simulink model "TOAD_Simulation_CPP"  (R2026a)
settings: Solver=VariableStepAuto  StopTime=50
values from neighbouring files (symbols this model uses):
  bGrom = G.C / (2 * sqrt(kGrom * m_FC))    [LoadTOADSim.m]
  constants6DoF = LoadTOADParams(Vehicle)    [LoadTOADSim.m]
  dt_SIM = 1/500    (= 0.002)    [LoadTOADSim.m]
  G_RMAX = 4    [LoadTOADSim.m]
  highEnd = 800    [LoadTOADSim.m]
  IMU_Rate = 500    [LoadTOADSim.m]
  Kg2 = 0.03    [LoadTOADSim.m]
  kGrom = G.K    [LoadTOADSim.m]
  lowEnd = 50    [LoadTOADSim.m]
  magDistMatrix = [dM_xx, dM_xy, dM_xz ... (first row only)    [LoadTOADSim.m]
  x0 = [1; zeros(12,1); constants6DoF.OxMass; constants6DoF.FuMass]    [LoadTOADSim.m]
undefined symbols (not defined in the file or in its folder): DiscIntNeverNeededParam, dt
libraries: aerolibnav x2, simulink x2
settings Model: PacingRate=0.890000  Creator=antho  LastModifiedBy=pplat

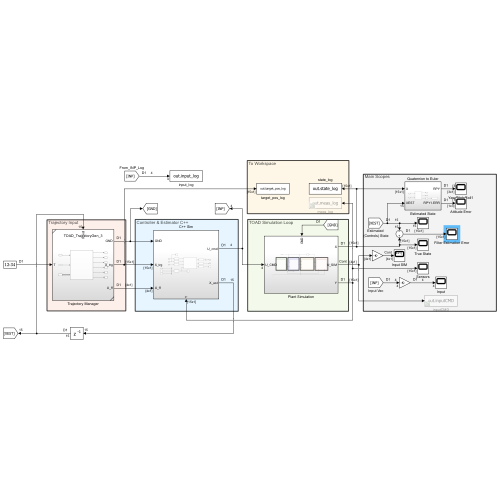
[thumbnail: Simulink's stored preview of the top-level diagram]
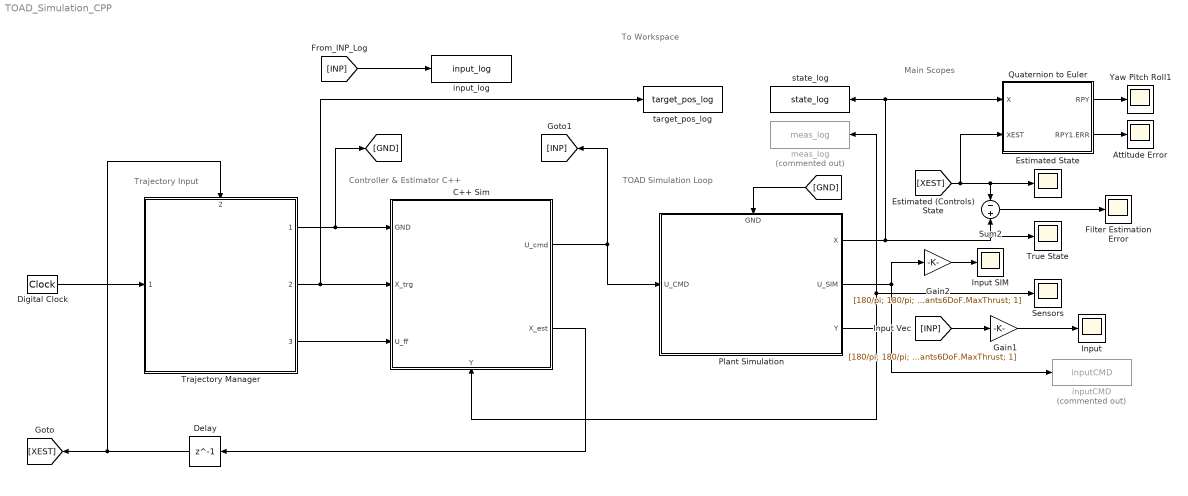
== system TOAD_Simulation_CPP ==
  note: To Workspace
  note: Main Scopes
  note: Trajectory Input
  note: Controller & Estimator C++
  note: TOAD Simulation Loop
  Attitude Error : Scope
      settings: ActiveDisplayYMinimum=-2.8585138814503157  ActiveDisplayYMaximum=11.108081672047327  DataLoggingVariableName=ScopeData9
  C++ Sim : Subsystem
      settings: PortSchema="{\"entries\":[{\"content\":{\"sides\":[{\"content\":{\"connectorIds\":[\"In1\",\"In2\",\"In3\"]},\"type\":\"ConnectorPlacement.EquallySpacedRectSide\",\"uuid\":\"4671e83a-8ca8-4575-bcdb-bf09507d43ac\"},{\"content\":{\"connectorIds\":[\"Out1\",\"Out2\"],\"side\":\"RIGHT\"},\"type\":\"ConnectorPlacement.EquallySpacedRectSide\",\"uuid\":\"a3e587af-0321-4bb5-b0a1-9da4dd43c686\"},{\"content\":{\"side\":\"TOP\"},\"type\":\"ConnectorPlacement.EquallySpacedRectSide\",\"uuid\":\"4e506283-964c-4194-bd88-e6573f16e4a7\"},{\"content\":{\"connectorIds\":[\"In4\"],\"side\":\"BOTTOM\"},\"type\":\"ConnectorPlacement.EquallySpacedRectSide\",\"uuid\":\"96ffffcd-a794-471a-8d82-32f73f1e6258\"}]},\"type\":\"ConnectorPlacement.EquallySpacedConnector\",\"uuid\":\"7e610c41-1f3b-432e-89ab-1ded86d82775\"}],\"packageUris\":[\"http://schema.mathworks.com/mf0/Connector/R2020b\"],\"version\":\"1.0\"}"
  Delay : Delay  DelayLength=1  InitialCondition=[1; zeros(14,1)]
  Digital Clock : DigitalClock  SampleTime=dt_SIM
  Estimated State : Scope
      settings: ActiveDisplayYMinimum=-0.79048423235500387  ActiveDisplayYMaximum=0.44471004558217864
  Filter Estimation Error : Scope
      settings: ActiveDisplayYMinimum=-0.43763268691917351  ActiveDisplayYMaximum=0.34444045907476623  DataLoggingVariableName=ScopeData2
  Gain1 : Gain  Gain=[180/pi; 180/pi; 1 / constants6DoF.MaxThrust; 1]
  Gain2 : Gain  Gain=[180/pi; 180/pi; 1 / constants6DoF.MaxThrust; 1]
  Input : Scope
      settings: ActiveDisplayYMinimum=-2.2667092424589841  ActiveDisplayYMaximum=2.729210355412238  DataLoggingVariableName=ScopeData6
  Input SIM : Scope
      settings: ActiveDisplayYMinimum=-2.0167562812566757  ActiveDisplayYMaximum=7.29010234773159  DataLoggingVariableName=ScopeData4
  Plant Simulation : Subsystem
      settings: PortSchema="{\"entries\":[{\"content\":{\"sides\":[{\"content\":{\"connectorIds\":[\"In1\"]},\"type\":\"ConnectorPlacement.EquallySpacedRectSide\",\"uuid\":\"1e23e861-4363-4f64-8b24-83286696985d\"},{\"content\":{\"connectorIds\":[\"Out1\",\"Out2\",\"Out3\"],\"side\":\"RIGHT\"},\"type\":\"ConnectorPlacement.EquallySpacedRectSide\",\"uuid\":\"b75b2d72-241b-467f-aafa-6008c8f1cd07\"},{\"content\":{\"connectorIds\":[\"In2\"],\"side\":\"TOP\"},\"type\":\"ConnectorPlacement.EquallySpacedRectSide\",\"uuid\":\"dda51a79-77a4-44ba-8754-0dda6b153588\"}]},\"type\":\"ConnectorPlacement.EquallySpacedConnector\",\"uuid\":\"1bd609f5-eeaa-4870-8a50-1642b8d6b239\"}],\"packageUris\":[\"http://schema.mathworks.com/mf0/Connector/R2020b\"],\"version\":\"1.0\"}"
  Quaternion to Euler : Subsystem
  Sensors : Scope
      settings: ActiveDisplayYMinimum=-0.86115231127145009  ActiveDisplayYMaximum=0.76236237160727249  DataLoggingVariableName=ScopeData3
  Sum2 : Sum  Inputs=-|+
  Trajectory Manager : Subsystem  ReferencedSubsystem=TOAD_TrajectoryGen_3
      settings: PortSchema="{\"entries\":[{\"content\":{\"sides\":[{\"content\":{\"connectorIds\":[\"In1\"]},\"type\":\"ConnectorPlacement.EquallySpacedRectSide\",\"uuid\":\"53aeece0-39f7-4f67-ba76-7d162a9bdc19\"},{\"content\":{\"connectorIds\":[\"Out1\",\"Out2\",\"Out3\"],\"side\":\"RIGHT\"},\"type\":\"ConnectorPlacement.EquallySpacedRectSide\",\"uuid\":\"ed850121-4575-4d77-9468-bb12120e9ba8\"},{\"content\":{\"connectorIds\":[\"In2\"],\"side\":\"TOP\"},\"type\":\"ConnectorPlacement.EquallySpacedRectSide\",\"uuid\":\"a0a50c51-23a8-460d-b4f4-86ce8b2346c6\"}]},\"type\":\"ConnectorPlacement.EquallySpacedConnector\",\"uuid\":\"ca42ea5e-ce10-4bee-86cd-a79e465aaa56\"}],\"packageUris\":[\"http://schema.mathworks.com/mf0/Connector/R2020b\"],\"version\":\"1.0\"}"
  True State : Scope
      settings: ActiveDisplayYMinimum=-0.82145720567291391  ActiveDisplayYMaximum=0.0015477167542865544
  Yaw Pitch Roll1 : Scope
      settings: ActiveDisplayYMinimum=-35.86119806852372  ActiveDisplayYMaximum=29.416743225810393  DataLoggingVariableName=ScopeData5
  inputCMD : ToWorkspace  Commented=on  VariableName=inputCMD  SaveFormat=Timeseries  SampleTime=-1
  input_log : ToWorkspace  VariableName=input_log  SaveFormat=Timeseries  SampleTime=0.02
  meas_log : ToWorkspace  Commented=on  VariableName=meas_log  SaveFormat=Timeseries  SampleTime=-1
  state_log : ToWorkspace  VariableName=state_log  SaveFormat=Timeseries  SampleTime=0.02
  target_pos_log : ToWorkspace  VariableName=target_pos_log  SaveFormat=Timeseries  SampleTime=0.02
  wires:
  Digital Clock/1 -> Trajectory Manager/1
  [XEST] -> Estimated State/1, Sum2/1, Quaternion to Euler/2(XEST)
  Sum2/1 -> Filter Estimation Error/1
  Trajectory Manager/1 -> [GND], C++ Sim/1(GND)
  [INP] -> Gain1/1
  Gain1/1 -> Input/1
  Gain2/1 -> Input SIM/1
  Plant Simulation/2(U_SIM) -> Gain2/1, inputCMD/1
  Plant Simulation/3(Y) -> C++ Sim/4(Y), meas_log/1, Sensors/1
  Plant Simulation/1(X) -> state_log/1, Quaternion to Euler/1(X), Sum2/2, True State/1
  Delay/1 -> Trajectory Manager/2, [XEST]
  Trajectory Manager/2 -> target_pos_log/1, C++ Sim/2(X_trg)
  Quaternion to Euler/1(RPY) -> Yaw Pitch Roll1/1
  Quaternion to Euler/2(RPY1.ERR) -> Attitude Error/1
  [GND] -> Plant Simulation/2(GND)
  [INP] -> input_log/1
  C++ Sim/1(U_cmd) -> Plant Simulation/1(U_CMD), [INP]
  Trajectory Manager/3 -> C++ Sim/3(U_ff)
  C++ Sim/2(X_est) -> Delay/1

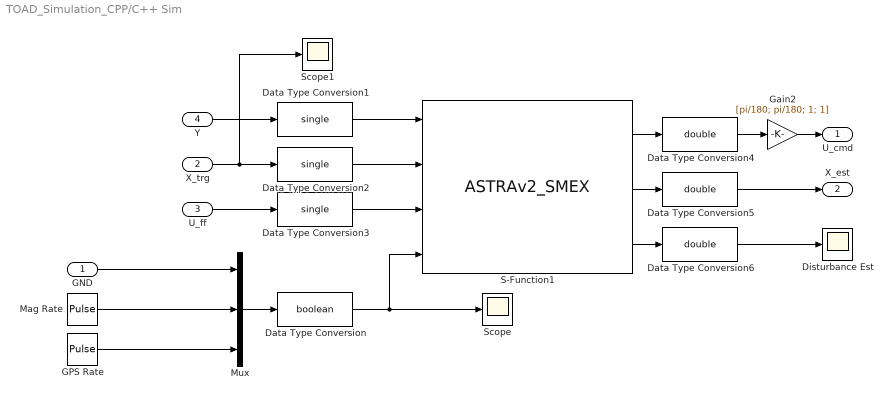
== system TOAD_Simulation_CPP/C++ Sim ==
  GND : Inport
  X_trg : Inport  Port=2
  U_ff : Inport  Port=3
  Y : Inport  Port=4
  Data Type Conversion : DataTypeConversion  OutDataTypeStr=boolean  SaturateOnIntegerOverflow=off  RndMeth=Floor
  Data Type Conversion1 : DataTypeConversion  OutDataTypeStr=single  SaturateOnIntegerOverflow=off  RndMeth=Floor
  Data Type Conversion2 : DataTypeConversion  OutDataTypeStr=single  SaturateOnIntegerOverflow=off  RndMeth=Floor
  Data Type Conversion3 : DataTypeConversion  OutDataTypeStr=single  SaturateOnIntegerOverflow=off  RndMeth=Floor
  Data Type Conversion4 : DataTypeConversion  OutDataTypeStr=double  SaturateOnIntegerOverflow=off  RndMeth=Floor
  Data Type Conversion5 : DataTypeConversion  OutDataTypeStr=double  SaturateOnIntegerOverflow=off  RndMeth=Floor
  Data Type Conversion6 : DataTypeConversion  OutDataTypeStr=double  SaturateOnIntegerOverflow=off  RndMeth=Floor
  Disturbance Est : Scope
      settings: ActiveDisplayYMinimum=-1  ActiveDisplayYMaximum=1  DataLoggingVariableName=ScopeData8
  GPS Rate : DiscretePulseGenerator  Period=50  SampleTime=dt_SIM
  Gain2 : Gain  Gain=[pi/180; pi/180; 1; 1]
  Mag Rate : DiscretePulseGenerator  Period=4  SampleTime=dt_SIM
  Mux : Mux  Inputs=3
  S-Function1 : S-Function  FunctionName=ASTRAv2_SMEX  SFunctionDeploymentMode=off  EnableBusSupport=off
  Scope : Scope
      settings: ActiveDisplayYMinimum=-0.12499999999999997  ActiveDisplayYMaximum=1.125  DataLoggingVariableName=ScopeData7
  Scope1 : Scope
      settings: ActiveDisplayYMinimum=-1  ActiveDisplayYMaximum=1  DataLoggingVariableName=ScopeData11
  U_cmd : Outport
  X_est : Outport  Port=2
  wires:
  S-Function1/2 -> Data Type Conversion5/1
  Y/1 -> Data Type Conversion1/1
  X_trg/1 -> Scope1/1, Data Type Conversion2/1
  S-Function1/1 -> Data Type Conversion4/1
  U_ff/1 -> Data Type Conversion3/1
  GND/1 -> Mux/1
  Mux/1 -> Data Type Conversion/1
  Mag Rate/1 -> Mux/2
  GPS Rate/1 -> Mux/3
  Data Type Conversion/1 -> Scope/1, S-Function1/4
  Data Type Conversion1/1 -> S-Function1/1
  Data Type Conversion2/1 -> S-Function1/2
  Data Type Conversion3/1 -> S-Function1/3
  Data Type Conversion4/1 -> Gain2/1
  Data Type Conversion5/1 -> X_est/1
  Gain2/1 -> U_cmd/1
  Data Type Conversion6/1 -> Disturbance Est/1
  S-Function1/3 -> Data Type Conversion6/1

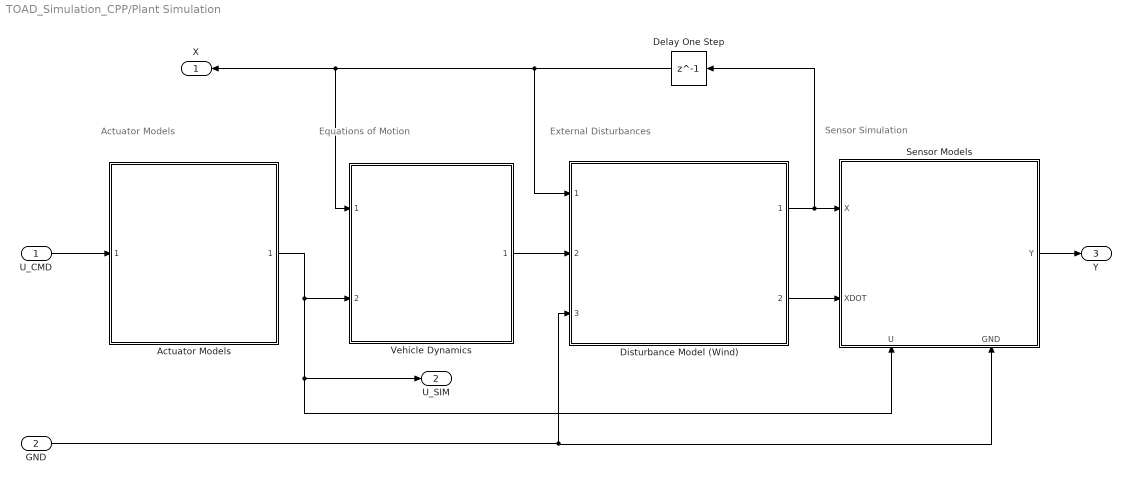
== system TOAD_Simulation_CPP/Plant Simulation ==
  note: Equations of Motion
  note: Actuator Models
  note: External Disturbances
  note: Sensor Simulation
  U_CMD : Inport
  GND : Inport  Port=2
  Actuator Models : Subsystem  ReferencedSubsystem=Actuator_Models_2
  Delay One Step : Delay  DelayLength=1  InitialCondition=x0
  Disturbance Model (Wind) : Subsystem  ReferencedSubsystem=Dist_Models_Integrator_2
  Sensor Models : Subsystem
      settings: PortSchema="{\"entries\":[{\"content\":{\"sides\":[{\"content\":{\"connectorIds\":[\"In1\",\"In2\"]},\"type\":\"ConnectorPlacement.EquallySpacedRectSide\",\"uuid\":\"9bc4a206-bba4-4c50-88a9-89b0392ab722\"},{\"content\":{\"connectorIds\":[\"Out1\"],\"side\":\"RIGHT\"},\"type\":\"ConnectorPlacement.EquallySpacedRectSide\",\"uuid\":\"162bbd17-e1b8-4f29-9191-53e17e38d79d\"},{\"content\":{\"side\":\"TOP\"},\"type\":\"ConnectorPlacement.EquallySpacedRectSide\",\"uuid\":\"c56a23db-6a5c-435f-99fd-d50fc9dbdc94\"},{\"content\":{\"connectorIds\":[\"In3\",\"In4\"],\"side\":\"BOTTOM\"},\"type\":\"ConnectorPlacement.EquallySpacedRectSide\",\"uuid\":\"e0c2a0dc-3b7a-40ac-8345-28e7bf7b9405\"}]},\"type\":\"ConnectorPlacement.EquallySpacedConnector\",\"uuid\":\"d1c29f55-9be5-4f45-9d70-06beba2c2f44\"}],\"packageUris\":[\"http://schema.mathworks.com/mf0/Connector/R2020b\"],\"version\":\"1.0\"}"
  Vehicle Dynamics : Subsystem  ReferencedSubsystem=Vehicle_Dynamics_2
  X : Outport
  U_SIM : Outport  Port=2
  Y : Outport  Port=3
  wires:
  Sensor Models/1(Y) -> Y/1
  Disturbance Model (Wind)/1 -> Delay One Step/1, Sensor Models/1(X)
  Disturbance Model (Wind)/2 -> Sensor Models/2(XDOT)
  Actuator Models/1 -> Vehicle Dynamics/2, U_SIM/1, Sensor Models/3(U)
  Vehicle Dynamics/1 -> Disturbance Model (Wind)/2
  U_CMD/1 -> Actuator Models/1
  GND/1 -> Disturbance Model (Wind)/3, Sensor Models/4(GND)
  Delay One Step/1 -> Disturbance Model (Wind)/1, Vehicle Dynamics/1, X/1

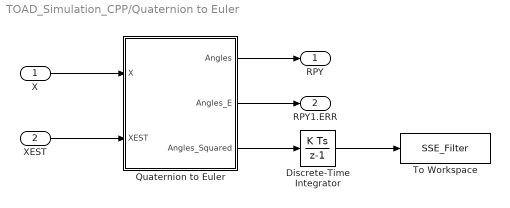
== system TOAD_Simulation_CPP/Quaternion to Euler ==
  X : Inport
  XEST : Inport  Port=2
  Discrete-Time Integrator : DiscreteIntegrator  InitialCondition=[0; 0; 0]'  SampleTime=-1  ICPrevOutput=DiscIntNeverNeededParam  ICPrevScaledInput=DiscIntNeverNeededParam
  Quaternion to Euler : MATLAB Function  TreatAsAtomicUnit=on
  To Workspace : ToWorkspace  VariableName=SSE_Filter  SampleTime=-1
      settings: MaxDataPoints=1
  RPY : Outport
  RPY1.ERR : Outport  Port=2
  wires:
  X/1 -> Quaternion to Euler/1(X)
  Quaternion to Euler/1(Angles) -> RPY/1
  XEST/1 -> Quaternion to Euler/2(XEST)
  Quaternion to Euler/2(Angles_E) -> RPY1.ERR/1
  Quaternion to Euler/3(Angles_Squared) -> Discrete-Time Integrator/1
  Discrete-Time Integrator/1 -> To Workspace/1

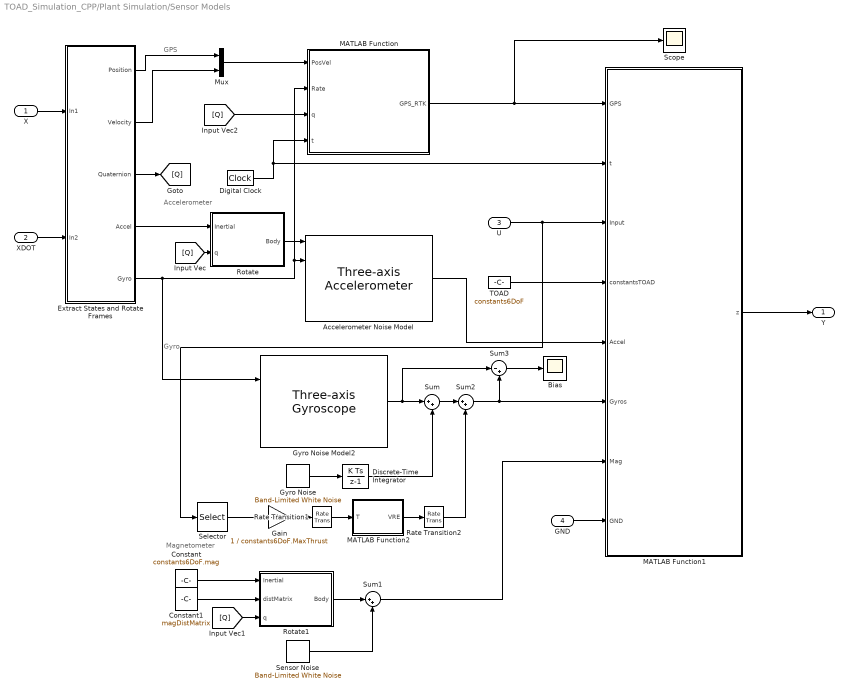
== system TOAD_Simulation_CPP/Plant Simulation/Sensor Models ==
  note: Gyro
  note: Accelerometer
  note: Magnetometer
  note: GPS
  X : Inport  PortDimensions=[15,1]
  XDOT : Inport  Port=2  PortDimensions=[15,1]
  U : Inport  Port=3
  GND : Inport  Port=4
  Accelerometer Noise Model : aerolibnav/Three-axis Accelerometer  units=Metric (MKS)  acc=[0 0 0.15]  gtype=on  dtype_a=on  w_a=190  z_a=0.707  a_sf_cc=eye(3)  a_bias=accelBias  a_Ts=1 / IMU_Rate  a_rand=on  a_seeds=[23093 23094 23095]  a_pow=ones(1,3) * 0.008^2 * 1 / IMU_Rate  a_sat="[-inf  -inf  -inf  inf inf inf]"
  Bias : Scope
      settings: ActiveDisplayYMinimum=-0.13135966855304979  ActiveDisplayYMaximum=1.1258739508928557  DataLoggingVariableName=ScopeData20
  Constant : Constant  Value=constants6DoF.mag
  Constant1 : Constant  Value=magDistMatrix
  Digital Clock : DigitalClock  SampleTime=dt_SIM
  Discrete-Time Integrator : DiscreteIntegrator  SampleTime=-1  ICPrevOutput=DiscIntNeverNeededParam  ICPrevScaledInput=DiscIntNeverNeededParam
  Extract States and Rotate Frames : Subsystem
  Gain : Gain  Gain=1 / constants6DoF.MaxThrust
  Gyro Noise : simulink/Sources/Band-Limited White Noise  Cov=gyroNoisePower  Ts=dt_SIM  seed=[23341,23342,23343]
  Gyro Noise Model2 : aerolibnav/Three-axis Gyroscope  dtype_g=on  w_g=190  z_g=0.707  g_sf_cc=eye(3)  g_bias=gyroBias  g_sen=0  g_Ts=1 / IMU_Rate  g_rand=on  g_seeds=[23093 23094 23095]  g_pow=ones(1,3) * 0.001^2 * dt  g_sat="[-inf  -inf  -inf  inf inf inf]"
  MATLAB Function : MATLAB Function  TreatAsAtomicUnit=on
  MATLAB Function1 : MATLAB Function  TreatAsAtomicUnit=on
  MATLAB Function2 : MATLAB Function  TreatAsAtomicUnit=on
  Mux : Mux  Inputs=2
  Rate Transition1 : RateTransition  InitialCondition=1  OutPortSampleTime=1/50
  Rate Transition2 : RateTransition  InitialCondition=1  OutPortSampleTime=dt_SIM
  Rotate : MATLAB Function  TreatAsAtomicUnit=on
  Rotate1 : MATLAB Function  TreatAsAtomicUnit=on
  Scope : Scope
      settings: ActiveDisplayYMinimum=-1  ActiveDisplayYMaximum=1  DataLoggingVariableName=ScopeData10
  Selector : Selector  IndexOptions=Index vector (dialog)  Indices=[3]  OutputSizes=1
  Sensor Noise : simulink/Sources/Band-Limited White Noise  Cov=(4E-4)^2  Ts=dt_SIM  seed=[23341,23342,23343]
  Sum : Sum  Inputs=|++
  Sum1 : Sum  Inputs=|++
  Sum2 : Sum  Inputs=|++
  Sum3 : Sum  Inputs=|-+
  TOAD : Constant  Value=constants6DoF  OutDataTypeStr=Bus: Vehicle_Bus
  Y : Outport
  wires:
  X/1 -> Extract States and Rotate Frames/1(In1)
  XDOT/1 -> Extract States and Rotate Frames/2(In2)
  Digital Clock/1 -> MATLAB Function/4(t), MATLAB Function1/2(t)
  Extract States and Rotate Frames/5(Gyro) -> Accelerometer Noise Model/2, MATLAB Function/2(Rate), Gyro Noise Model2/1
  Extract States and Rotate Frames/3(Quaternion) -> [Q]
  Rotate/1(Body) -> Accelerometer Noise Model/1
  Extract States and Rotate Frames/4(Accel) -> Rotate/1(Inertial)
  [Q] -> Rotate/2(q)
  Constant/1 -> Rotate1/1(Inertial)
  [Q] -> Rotate1/3(q)
  Sensor Noise/1 -> Sum1/2
  Rotate1/1(Body) -> Sum1/1
  Sum1/1 -> MATLAB Function1/7(Mag)
  MATLAB Function/1(GPS_RTK) -> Scope/1, MATLAB Function1/1(GPS)
  Accelerometer Noise Model/1 -> MATLAB Function1/5(Accel)
  Gyro Noise Model2/1 -> Sum3/1, Sum/1
  MATLAB Function1/1(z) -> Y/1
  TOAD/1 -> MATLAB Function1/4(constantsTOAD)
  Extract States and Rotate Frames/2(Velocity) -> Mux/2
  Mux/1 -> MATLAB Function/1(PosVel)
  Extract States and Rotate Frames/1(Position) -> Mux/1
  U/1 -> Selector/1, MATLAB Function1/3(Input)
  GND/1 -> MATLAB Function1/8(GND)
  Constant1/1 -> Rotate1/2(distMatrix)
  [Q] -> MATLAB Function/3(q)
  Gyro Noise/1 -> Discrete-Time Integrator/1
  Sum/1 -> Sum2/1
  Discrete-Time Integrator/1 -> Sum/2
  MATLAB Function2/1(VRE) -> Rate Transition2/1
  Sum2/1 -> MATLAB Function1/6(Gyros), Sum3/2
  Selector/1 -> Gain/1
  Gain/1 -> Rate Transition1/1
  Sum3/1 -> Bias/1
  Rate Transition1/1 -> MATLAB Function2/1(T)
  Rate Transition2/1 -> Sum2/2

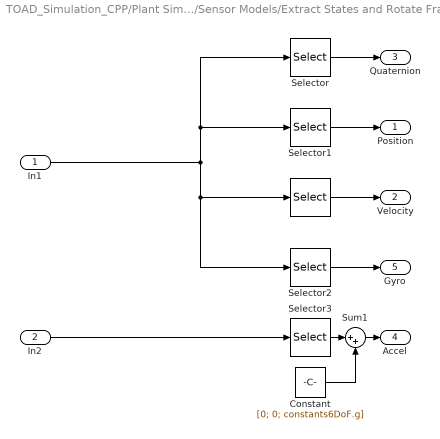
== system TOAD_Simulation_CPP/Plant Simulation/Sensor Models/Extract States and Rotate Frames ==
  In1 : Inport
  In2 : Inport  Port=2
  "  " : Selector  IndexOptions=Index vector (dialog)  Indices=[8:10]  OutputSizes=1
  Constant : Constant  Value=[0; 0; constants6DoF.g]
  Selector : Selector  IndexOptions=Index vector (dialog)  Indices=[1:4]  OutputSizes=1
  Selector1 : Selector  IndexOptions=Index vector (dialog)  Indices=[5:7]  OutputSizes=1
  Selector2 : Selector  IndexOptions=Index vector (dialog)  Indices=[11:13]  OutputSizes=1
  Selector3 : Selector  IndexOptions=Index vector (dialog)  Indices=[8:10]  OutputSizes=1
  Sum1 : Sum  Inputs=|++
  Position : Outport
  Velocity : Outport  Port=2
  Quaternion : Outport  Port=3
  Accel : Outport  Port=4
  Gyro : Outport  Port=5
  wires:
  Selector/1 -> Quaternion/1
  Selector1/1 -> Position/1
  "  "/1 -> Velocity/1
  Selector2/1 -> Gyro/1
  Selector3/1 -> Sum1/1
  Sum1/1 -> Accel/1
  Constant/1 -> Sum1/2
  In1/1 -> Selector1/1, Selector/1, Selector2/1, "  "/1
  In2/1 -> Selector3/1

== matlab function TOAD_Simulation_CPP/Quaternion to Euler/Quaternion to Euler ==
  data: X input; Angles output; XEST input; Angles_E output; Angles_Squared output
function [Angles, Angles_E, Angles_Squared] = q2eul(X, XEST)

% Complete quaternion & error quaternion
q = X(1:4);
qest = XEST(1:4);

Q_Conj = [qest(1); -qest(2:4)];
qerr = HamiltonianProd(Q_Conj) * q;
if qerr(1) < 0
    qerr = -qerr;
end

% Quaternion to Euler Angles
Roll = atan2(2*(q(1) * q(2) + q(3) * q(4)), 1 - 2*(q(2)^2 + q(3)^2));
Pitch = asin(2*(q(1) * q(3) - q(4) * q(2)));
Yaw = atan2(2*(q(1) * q(4) + q(2) * q(3)), 1 - 2*(q(3)^2 + q(4)^2));

% Error Euler Angles
Roll_E = atan2(2*(qerr(1) * qerr(2) + qerr(3) * qerr(4)), 1 - 2*(qerr(2)^2 + qerr(3)^2));
Pitch_E = asin(2*(qerr(1) * qerr(3) - qerr(4) * qerr(2)));
Yaw_E = atan2(2*(qerr(1) * qerr(4) + qerr(2) * qerr(3)), 1 - 2*(qerr(3)^2 + qerr(4)^2));

% Angle Vector
Angles = [Roll; Pitch; Yaw] * 180/pi;
Angles_E = [Roll_E; Pitch_E; Yaw_E]' * 180/pi;
Angles_Squared = Angles_E.^2;

== matlab function TOAD_Simulation_CPP/Plant Simulation/Sensor Models/MATLAB Function2 ==
  data: T input; VRE output; G_RMAX parameter; kGrom parameter; bGrom parameter; Kg2 parameter; lowEnd parameter; highEnd parameter
function VRE = VRECalc(T, G_RMAX, kGrom, bGrom, Kg2, lowEnd, highEnd)
    VRE = VRECalc(T, G_RMAX, kGrom, bGrom, Kg2, lowEnd, highEnd);

== matlab function TOAD_Simulation_CPP/Plant Simulation/Sensor Models/Rotate ==
  data: Inertial input; Body output; q input
function Body = Rotate(Inertial, q)
Body = quatRot(q) * Inertial;

== matlab function TOAD_Simulation_CPP/Plant Simulation/Sensor Models/Rotate1 ==
  data: Inertial input; distMatrix input; Body output; q input
function Body = Rotate(Inertial, distMatrix, q)

Scale = 0.51993;
Body = (distMatrix * (quatRot(q) * Inertial) + [0.01; 0.01; 0.005]) * Scale;

== matlab function TOAD_Simulation_CPP/Plant Simulation/Sensor Models/MATLAB Function ==
  data: PosVel input; Rate input; q input; GPS_RTK output; t input
function GPS_RTK = GPS(PosVel, Rate, q, t)

R_b2i = quatRot(q)';
GPS_RTK = GPS_Sim(PosVel, Rate, R_b2i, t);

== matlab function TOAD_Simulation_CPP/Plant Simulation/Sensor Models/MATLAB Function1 ==
  settings: updateMethod=DISCRETE
  data: GPS input; t input; Input input; constantsTOAD input; Accel input; z output; Gyros input; Mag input; GND input
function z = SensorFrequency(GPS, t, Input, constantsTOAD, Accel, Gyros, Mag, GND)
%% Add Thrust Varying Oscillation
persistent phase lastT
if isempty(phase)
    phase = 0;
    lastT = 0;
end
dt = t - lastT;
lastT = t;

% Thrust vibration generator
Track = [1.3525    42.6278];
THRUST = Input(3) / constantsTOAD.MaxThrust * 100;
w = 2 * pi * (Track(1) * THRUST + Track(2) + 1 * randn());
phase = phase + w * dt;
MaxAmplAccel = 7;
MaxAmplGyro = 0.2;
Accel = Accel + MaxAmplAccel * THRUST / 100 * sin(phase) * (1 - GND);
Gyros = Gyros + MaxAmplGyro * THRUST / 100 * sin(phase) * (1 - GND);
z = [Accel; Gyros; Mag; GPS];
